simulink model "PLLKnownInput"  (R2025b)
settings: Solver=FixedStepDiscrete  StartTime=0.0  StopTime=.6  FixedStep=1e-6  RelTol=1e-3
model workspace (MAT data in the model file):
  pllInput = [0 1e-06 2e-06 3e-06 4e-06 5e-06 6e-06 7e-06 8e-06 9e-06 1e-05 1.1e-05 ... (2400004 elements, 600001x4)]
libraries: eeSinusoidalMeasurement x1
settings Model: Creator=18483  LastModifiedBy=18483
settings DataIOCC: SaveOutput=off  SaveTime=off

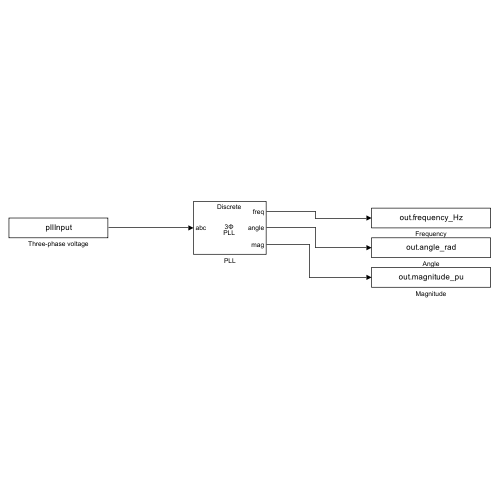
[thumbnail: Simulink's stored preview of the top-level diagram]
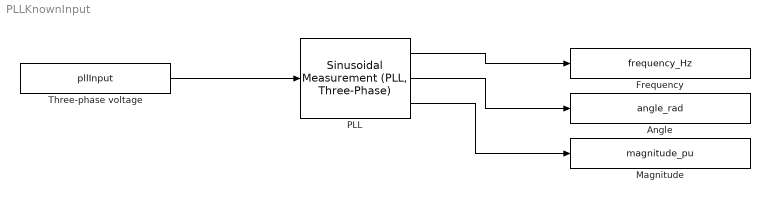
== system PLLKnownInput ==
  Angle : ToWorkspace  VariableName=angle_rad  SaveFormat=Timeseries  SampleTime=-1
  Frequency : ToWorkspace  VariableName=frequency_Hz  SaveFormat=Timeseries  SampleTime=-1
  Magnitude : ToWorkspace  VariableName=magnitude_pu  SaveFormat=Timeseries  SampleTime=-1
  PLL : eeSinusoidalMeasurement/Sinusoidal Measurement (PLL, Three-Phase)  Kp_LF=180  Ki_LF=3200  F0=50  Theta0=0  Ts=1e-6
  Three-phase voltage : FromWorkspace  VariableName=pllInput
  wires:
  Three-phase voltage/1 -> PLL/1
  PLL/1 -> Frequency/1
  PLL/2 -> Angle/1
  PLL/3 -> Magnitude/1
